simulink model "wind"  (R2025b)
settings: Solver=ode45  StartTime=0.0  StopTime=10  RelTol=1e-3
undefined symbols (not defined in the file): P
settings Model: Creator=parakh  LastModifiedBy=parakh

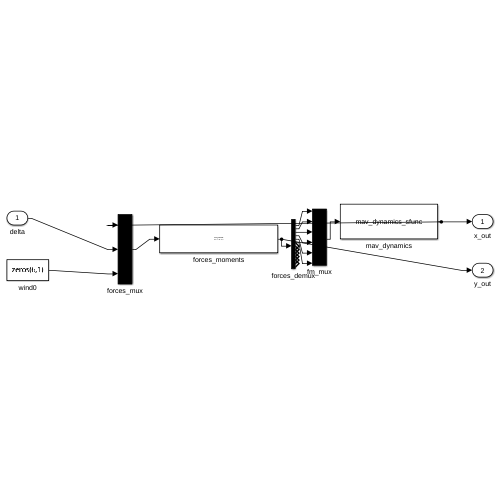
[thumbnail: Simulink's stored preview of the top-level diagram]
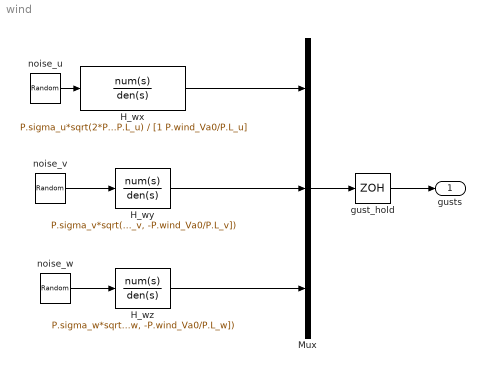
== system wind ==
  H_wx : TransferFcn  Numerator=P.sigma_u*sqrt(2*P.wind_Va0/P.L_u)  Denominator=[1 P.wind_Va0/P.L_u]
  H_wy : TransferFcn  Numerator=P.sigma_v*sqrt(3*P.wind_Va0/P.L_v)*[0, 1, P.wind_Va0/sqrt(3)/P.L_v]  Denominator=poly([-P.wind_Va0/P.L_v, -P.wind_Va0/P.L_v])
  H_wz : TransferFcn  Numerator=P.sigma_w*sqrt(3*P.wind_Va0/P.L_w)*[0, 1, P.wind_Va0/sqrt(3)/P.L_w]  Denominator=poly([-P.wind_Va0/P.L_w, -P.wind_Va0/P.L_w])
  Mux : Mux  Inputs=3
  noise_u : RandomNumber  SampleTime=0
  noise_v : RandomNumber  SampleTime=0
  noise_w : RandomNumber  SampleTime=0
  gust_hold : ZeroOrderHold  SampleTime=P.Ts
  gusts : Outport
  wires:
  H_wx/1 -> Mux/1
  noise_u/1 -> H_wx/1
  H_wy/1 -> Mux/2
  noise_v/1 -> H_wy/1
  H_wz/1 -> Mux/3
  noise_w/1 -> H_wz/1
  Mux/1 -> gust_hold/1
  gust_hold/1 -> gusts/1
